simulink model "SensoSpoon_Control"  (R2026a)
settings: Solver=ode23t  StopTime=4  MaxStep=.001  RelTol=1e-4  AbsTol=1e-6
model workspace (MAT data in the model file):
  B(1).mass = 0.00253187337457
  B(1).com = [0.000428308261577; -3.33592024592e-19; -1.28078157724e-20]
  B(1).inertia = [7.38028719368e-08  -3.07478426256e-25  -1.32817521062e-25; -3.07478426256e-25  1.0653311692e-08  -5.88805898006e-25; -1.32817521062e-25  -5.88805898006e-25  7.14205635889e-08]
  B(2).mass = 0.046143480036
  B(2).com = [-0.0497444579629; 4.45344279178e-08; -0.0071916014832]
  B(2).inertia = [4.24326445066e-06  6.29131950445e-12  -4.63292057823e-06; 6.29131950445e-12  4.58365200995e-05  4.90790351694e-11; -4.63292057823e-06  4.90790351694e-11  4.73513997823e-05]
  B(3).mass = 0.011
  B(3).com = [0.049; -0.005; 0.006]
  B(3).inertia = [1.98e-07  0  0; 0  2.31e-07  0; 0  0  2.31e-07]
  B(4).mass = 0.0127643184343
  B(4).com = [0.0761622058383; 0.005; 0.006]
  B(4).inertia = [1.99984858239e-07  0  0; 0  2.24509835442e-06  0; 0  0  2.24509835442e-06]
  B(5).mass = 0.000712000026889
  B(5).com = [0; 0; 0]
  B(5).inertia = [3.56000013445e-10  0  0; 0  5.02701685652e-08  0; 0  0  5.02701685652e-08]
  B(6).mass = 0.000712000026889
  B(6).com = [0; 0; 0]
  B(6).inertia = [3.56000013445e-10  0  0; 0  5.02701685652e-08  0; 0  0  5.02701685652e-08]
  Bnom(1).mass = 0.00253187337457
  Bnom(1).com = [0.000428308261577; -3.33592024592e-19; -1.28078157724e-20]
  Bnom(1).inertia = [7.38028719368e-08  -3.07478426256e-25  -1.32817521062e-25; -3.07478426256e-25  1.0653311692e-08  -5.88805898006e-25; -1.32817521062e-25  -5.88805898006e-25  7.14205635889e-08]
  Bnom(2).mass = 0.043143480036
  Bnom(2).com = [-0.0486280291057; 4.76311480628e-08; -0.0069963183131]
  Bnom(2).inertia = [4.11170784507e-06  8.58555120438e-12  -4.48824336546e-06; 8.58555120438e-12  4.48215975922e-05  4.94803369061e-11; -4.48824336546e-06  4.94803369061e-11  4.62680338807e-05]
  Bnom(3).mass = 0.011
  Bnom(3).com = [0.049; -0.005; 0.006]
  Bnom(3).inertia = [1.98e-07  0  0; 0  2.31e-07  0; 0  0  2.31e-07]
  Bnom(4).mass = 0.0127643184343
  Bnom(4).com = [0.0761622058383; 0.005; 0.006]
  Bnom(4).inertia = [1.99984858239e-07  0  0; 0  2.24509835442e-06  0; 0  0  2.24509835442e-06]
  Bnom(5).mass = 0.000712000026889
  Bnom(5).com = [0; 0; 0]
  Bnom(5).inertia = [3.56000013445e-10  0  0; 0  5.02701685652e-08  0; 0  0  5.02701685652e-08]
  Bnom(6).mass = 0.000712000026889
  Bnom(6).com = [0; 0; 0]
  Bnom(6).inertia = [3.56000013445e-10  0  0; 0  5.02701685652e-08  0; 0  0  5.02701685652e-08]
  C.outer_hz = 800
  C.current_hz = 10000
  C.intent_filter = 'notch'
  C.notch_frequencies_Hz = [4 6 8 10 12]
  C.notch_bandwidth_Hz = 7
  C.intent_lead_s = 0.14
  C.intent_lead_pole_Hz = 1
  C.intent_rolloff_Hz = 10
  C.intent_hz = 1
  C.complement_hz = 0.05
  C.natural_hz = 35
  C.damping = 0.85
  C.integral_gain = 80
  C.current_kp = 0.8
  C.current_ki = 2000
  C.current_aw = 1500
  C.joint_limit = 0.244346095279
  C.reference_rate = 3.14159265359
  C.gyro_bias = [0.00347103685272; -0.00265540804355; 0.00180286392436; 0.00338772797741; -0.00268367652419; 0.00171822476761]
  C.accel_bias = [0.0499265864944; -0.0791463213806; 0.0291179813156; 0.0494836591873; -0.0770543876801; 0.0282725288544]
  C.current_quantum = 0.001708984375
  C.current_offset = [0.001; -0.001]
  C.current_noise_A = 0.0005
  C.power_window_s = 2
  C.seed = 1701
  C.name = 'simple_pid'
  C.intent_sos = [0.97325077265  -1.94554106429  0.97325077265  1  -1.94554106429  0.946501545301; 0.973256125668  -1.94435137935  0.973256125668  1  -1.94435137935  0.946512251336; 0.973263618882  -1.9426862109  0.973263618882  1  -1.9426862109  0.946527237765; 0.973273251283  -1.94054594933  0.973273251283  1  -1.94054594933  0.946546502566; 0.973285021571  -1.93793109639  0.973285021571  1  -1.93793109639  0.946570043141; 1.87620507603  -1.86838177621  0  1  -0.992176700178  0; 0.00146031630553  0.00292063261106  0.00146031630553  1  -1.88903307939  0.894874344617]
  H.revision = 'RCFlex_curved_neck_v17'
  H.total_length_mm = 271
  H.handle_mm = [168 30 24]
  H.bowl_mm = [62 40 12]
  H.bowl_tip_x_mm = -103
  H.bowl_widest_station_mm = 37.2
  H.bowl_front_width_mm = 28
  H.bowl_front_station_mm = 10.6338862458
  H.bowl_connection_width_mm = 10
  H.bowl_bottom_thickness_mm = 1.8
  H.bowl_measurement_x_mm = -65.8
  H.bowl_rim_z_mm = -4
  H.neck_length_mm = 31
  H.gimbal_mm = [25 33 19]
  H.pushrod_diameter_mm = 2
  H.physical_travel_deg = 15
  H.grip_x_mm = 65
  H.remote_center_x_mm = NaN
  H.equivalent_center_x_mm = 0
  H.shell_wall_mm = 1.4
  H.shell_x_mm = [0 18 35 55 80 100 130 150 160 168]
  H.shell_y_scale = [1.4 1.33333333333 1.2 1.1 1.08666666667 1.10666666667 1.14666666667 1.08666666667 0.8 0.133333333333]
  H.shell_z_scale = [1.75 1.66666666667 1.48333333333 1.16666666667 1.125 1.16666666667 1.25 1.16666666667 0.916666666667 0.166666666667]
  H.shell_center_z_mm = [0 0 1.5 4 6 6 6 6 6 6]
  H.ball_outer_radius_mm = 17
  H.ball_inner_radius_mm = 16.2
  H.ball_x_limits_mm = [-15.5 -3]
  H.bezel_outer_radius_mm = 21
  H.bezel_inner_radius_mm = 19.8
  H.bezel_x_limits_mm = [-16 0]
  H.front_cap_x_mm = 18
  H.front_rod_windows_mm = [-6.5  -2  9  18; 6.5  -2  9  18]
  H.bowl_wall_mm = 1.2
  H.vca_length_mm = 23.9
  H.vca_diameter_mm = 15.9
  H.vca_centers_mm = [55.5  -5  6; 87.5  5  6]
  H.vca_stroke_mm = 6.35
  H.vca_force_peak_N = 4.6
  H.vca_force_cont_N = 1.5
  H.vca_force_constant_N_A = 1.5
  H.steel_E_Pa = 200000000000
  H.flexure_pivot_parts = {'C-Flex B-10 x2 (pitch)', 'C-Flex D-10 x1 (roll)'}
  H.flexure_stiffness_Nm_rad = [0.00517884308057; 0.0116523969313]
  H.flexure_stiffness_tolerance = 0.1
  H.flexure_damping_Nms_rad = 0.0002
  H.flexure_cubic_ratio = 0
  H.fs = 1000
  H.duration = 20
  H.link.pivot = [0.012  0.012; -0.005  0.005; 0.0075  0.0075]
  H.link.mode = 'direct'
  H.link.attachment = [0.006  0.006; -0.0085  0.0085; -0.01  -0.01]
  H.link.slider_x = [0.03 0.03]
  H.link.slider_z = 0.006
  H.link.input_length = [0.0290559804515 0.0290559804515]
  H.link.output_length = 0
  H.coil_R_ohm = 4.6
  H.coil_L_H = 0.0008
  H.bus_voltage_V = 7.4
  H.current_limit_A = 1.5
  H.coil_alpha_K = 0.00393
  H.coil_mass_kg = 0.011
  H.motor_body_mass_kg = 0.017
  H.coil_continuous_power_W = 4.4
  H.shaft_side_load_N = 2.2
  H.driver_R_ohm = 0.7
  H.driver_pwm_hz = 20000
  H.driver_min_voltage_V = 4.5
  H.battery_capacity_Ah = 0.4
  H.battery_R_ohm = 0.15
  H.battery_mass_kg = 0.018
  H.battery_mm = [41 20 13]
  H.motor_part = 'Moticont GVCM-016-019-01M'
  H.driver_part = 'TI DRV8876PWPR'
  H.guide_friction_N = 0.03
  H.guide_viscous_Ns_m = 0.03
  H.imu_part = 'Bosch BMI270'
  H.imu_gyro_noise_dps_sqrtHz = 0.007
  H.imu_acc_noise_g_sqrtHz = 0.00016
  H.imu_gyro_offset_dps = 0.5
  H.imu_rate_hz = 800
  H.ambient_C = 25
  H.thermal_capacity_J_K = 8
  H.thermal_resistance_K_W = 18
  H.stop_stiffness_Nm_rad = 8
  H.stop_damping_Nms_rad = 0.025
  H.slider_stop_N_m = 10000
  H.slider_stop_Ns_m = 2
  H.food_mass_kg = 0.008
  H.sensor_seed = 1701
  Hnom.revision = 'RCFlex_curved_neck_v17'
  Hnom.total_length_mm = 271
  Hnom.handle_mm = [168 30 24]
  Hnom.bowl_mm = [62 40 12]
  Hnom.bowl_tip_x_mm = -103
  Hnom.bowl_widest_station_mm = 37.2
  Hnom.bowl_front_width_mm = 28
  Hnom.bowl_front_station_mm = 10.6338862458
  Hnom.bowl_connection_width_mm = 10
  Hnom.bowl_bottom_thickness_mm = 1.8
  Hnom.bowl_measurement_x_mm = -65.8
  Hnom.bowl_rim_z_mm = -4
  Hnom.neck_length_mm = 31
  Hnom.gimbal_mm = [25 33 19]
  Hnom.pushrod_diameter_mm = 2
  Hnom.physical_travel_deg = 15
  Hnom.grip_x_mm = 65
  Hnom.remote_center_x_mm = NaN
  Hnom.equivalent_center_x_mm = 0
  Hnom.shell_wall_mm = 1.4
  Hnom.shell_x_mm = [0 18 35 55 80 100 130 150 160 168]
  Hnom.shell_y_scale = [1.4 1.33333333333 1.2 1.1 1.08666666667 1.10666666667 1.14666666667 1.08666666667 0.8 0.133333333333]
  Hnom.shell_z_scale = [1.75 1.66666666667 1.48333333333 1.16666666667 1.125 1.16666666667 1.25 1.16666666667 0.916666666667 0.166666666667]
  Hnom.shell_center_z_mm = [0 0 1.5 4 6 6 6 6 6 6]
  Hnom.ball_outer_radius_mm = 17
  Hnom.ball_inner_radius_mm = 16.2
  Hnom.ball_x_limits_mm = [-15.5 -3]
  Hnom.bezel_outer_radius_mm = 21
  Hnom.bezel_inner_radius_mm = 19.8
  Hnom.bezel_x_limits_mm = [-16 0]
  Hnom.front_cap_x_mm = 18
  Hnom.front_rod_windows_mm = [-6.5  -2  9  18; 6.5  -2  9  18]
  Hnom.bowl_wall_mm = 1.2
  Hnom.vca_length_mm = 23.9
  Hnom.vca_diameter_mm = 15.9
  Hnom.vca_centers_mm = [55.5  -5  6; 87.5  5  6]
  Hnom.vca_stroke_mm = 6.35
  Hnom.vca_force_peak_N = 4.6
  Hnom.vca_force_cont_N = 1.5
  Hnom.vca_force_constant_N_A = 1.5
  Hnom.steel_E_Pa = 200000000000
  Hnom.flexure_pivot_parts = {'C-Flex B-10 x2 (pitch)', 'C-Flex D-10 x1 (roll)'}
  Hnom.flexure_stiffness_Nm_rad = [0.00517884308057; 0.0116523969313]
  Hnom.flexure_stiffness_tolerance = 0.1
  Hnom.flexure_damping_Nms_rad = 0.0002
  Hnom.flexure_cubic_ratio = 0
  Hnom.fs = 1000
  Hnom.duration = 20
  Hnom.link.pivot = [0.012  0.012; -0.005  0.005; 0.0075  0.0075]
  Hnom.link.mode = 'direct'
  Hnom.link.attachment = [0.006  0.006; -0.0085  0.0085; -0.01  -0.01]
  Hnom.link.slider_x = [0.03 0.03]
  Hnom.link.slider_z = 0.006
  Hnom.link.input_length = [0.0290559804515 0.0290559804515]
  Hnom.link.output_length = 0
  Hnom.coil_R_ohm = 4.6
  Hnom.coil_L_H = 0.0008
  Hnom.bus_voltage_V = 7.4
  Hnom.current_limit_A = 1.5
  Hnom.coil_alpha_K = 0.00393
  Hnom.coil_mass_kg = 0.011
  Hnom.motor_body_mass_kg = 0.017
  Hnom.coil_continuous_power_W = 4.4
  Hnom.shaft_side_load_N = 2.2
  Hnom.driver_R_ohm = 0.7
  Hnom.driver_pwm_hz = 20000
  Hnom.driver_min_voltage_V = 4.5
  Hnom.battery_capacity_Ah = 0.4
  Hnom.battery_R_ohm = 0.15
  Hnom.battery_mass_kg = 0.018
  Hnom.battery_mm = [41 20 13]
  Hnom.motor_part = 'Moticont GVCM-016-019-01M'
  Hnom.driver_part = 'TI DRV8876PWPR'
  Hnom.guide_friction_N = 0.03
  Hnom.guide_viscous_Ns_m = 0.03
  Hnom.imu_part = 'Bosch BMI270'
  Hnom.imu_gyro_noise_dps_sqrtHz = 0.007
  Hnom.imu_acc_noise_g_sqrtHz = 0.00016
  Hnom.imu_gyro_offset_dps = 0.5
  Hnom.imu_rate_hz = 800
  Hnom.ambient_C = 25
  Hnom.thermal_capacity_J_K = 8
  Hnom.thermal_resistance_K_W = 18
  Hnom.stop_stiffness_Nm_rad = 8
  Hnom.stop_damping_Nms_rad = 0.025
  Hnom.slider_stop_N_m = 10000
  Hnom.slider_stop_Ns_m = 2
  Hnom.food_mass_kg = 0.005
  base_motion = timeseries
  base_motion.Name = 'unnamed'
  base_motion.DataInfo = tsdata.datametadata
  base_motion.DataInfo.Interpolation = tsdata.interpolation
  base_motion.DataInfo.Interpolation.Fhandle : function handle (value not decoded)
  base_motion.DataInfo.Interpolation.Name = 'linear'
  base_motion.TimeInfo = tsdata.timemetadata
  base_motion.TimeInfo.Length = 80001
  base_motion.TimeInfo.DuplicateTimes = 0
  base_motion.TimeInfo.Time_ = [0 5e-05 0.0001 0.00015 0.0002 0.00025 0.0003 0.00035 0.0004 0.00045 0.0005 0.00055 ... (80001 elements, 80001x1)]
  base_motion.TimeInfo.Initialized = 1
  base_motion.QualityInfo = tsdata.qualmetadata
  base_motion.Data_ = [0 0 0 0 0 0 0 0 0 0 0 0 ... (1200015 elements, 80001x15)]
  mode = 'voltage'
  voltage_command = timeseries
  voltage_command.Name = 'unnamed'
  voltage_command.DataInfo = tsdata.datametadata
  voltage_command.DataInfo.Interpolation = tsdata.interpolation
  voltage_command.DataInfo.Interpolation.Fhandle : function handle (value not decoded)
  voltage_command.DataInfo.Interpolation.Name = 'linear'
  voltage_command.TimeInfo = tsdata.timemetadata
  voltage_command.TimeInfo.Length = 6001
  voltage_command.TimeInfo.DuplicateTimes = 0
  voltage_command.TimeInfo.Time_ = [0 0.001 0.002 0.003 0.004 0.005 0.006 0.007 0.008 0.009 0.01 0.011 ... (6001 elements, 6001x1)]
  voltage_command.TimeInfo.Initialized = 1
  voltage_command.QualityInfo = tsdata.qualmetadata
  voltage_command.Data_ = [0 0 0 0 0 0 0 0 0 0 0 0 ... (12002 elements, 6001x2)]
settings Model: Creator=tomli  LastModifiedBy=Aditya

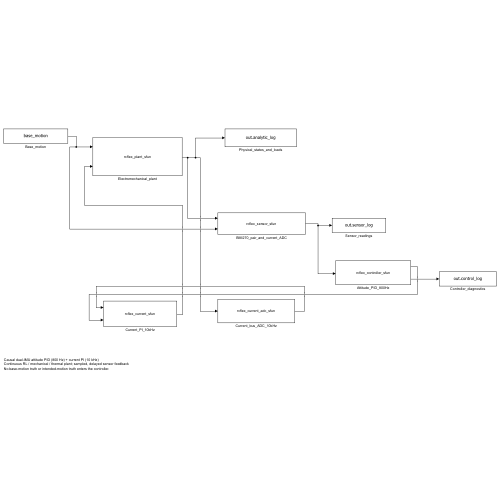
[thumbnail: Simulink's stored preview of the top-level diagram]
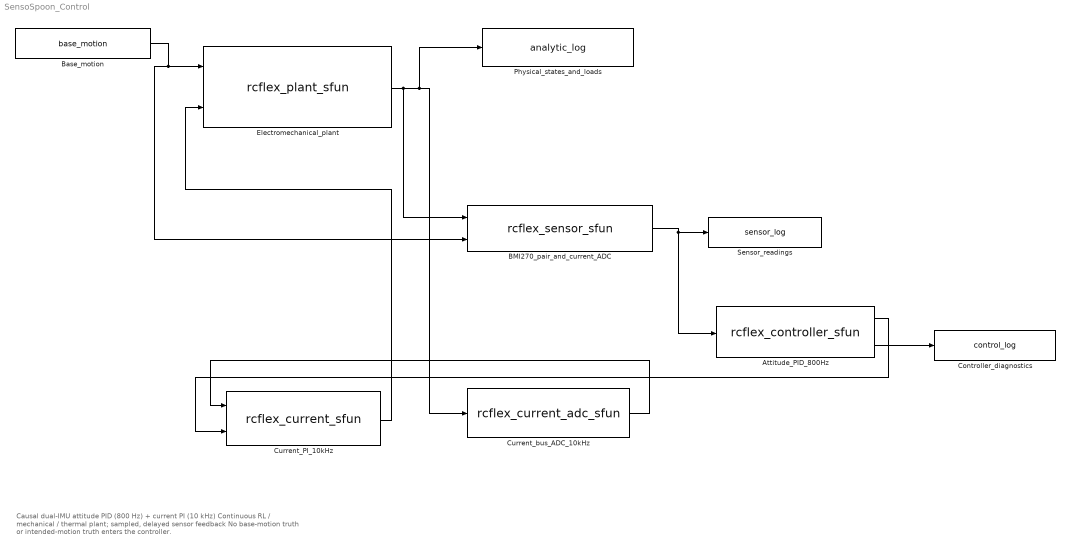
== system SensoSpoon_Control ==
  note: Causal dual-IMU attitude PID (800 Hz) + current PI (10 kHz)
      | Continuous RL / mechanical / thermal plant; sampled, delayed sensor feedback
      | No base-motion truth or intended-motion truth enters the controller.
  Attitude_PID_800Hz : M-S-Function  FunctionName=rcflex_controller_sfun  Parameters=Hnom,Bnom,C
  BMI270_pair_and_current_ADC : M-S-Function  FunctionName=rcflex_sensor_sfun  Parameters=H
  Base_motion : FromWorkspace  VariableName=base_motion
  Controller_diagnostics : ToWorkspace  VariableName=control_log  SaveFormat=Timeseries  SampleTime=-1
  Current_PI_10kHz : M-S-Function  FunctionName=rcflex_current_sfun  Parameters=Hnom,C
  Current_bus_ADC_10kHz : M-S-Function  FunctionName=rcflex_current_adc_sfun  Parameters=H,C
  Electromechanical_plant : M-S-Function  FunctionName=rcflex_plant_sfun  Parameters=H,B,mode
  Physical_states_and_loads : ToWorkspace  VariableName=analytic_log  SaveFormat=Timeseries  SampleTime=-1
  Sensor_readings : ToWorkspace  VariableName=sensor_log  SaveFormat=Timeseries  SampleTime=-1
  wires:
  Base_motion/1 -> BMI270_pair_and_current_ADC/2, Electromechanical_plant/1
  Electromechanical_plant/1 -> Physical_states_and_loads/1, Current_bus_ADC_10kHz/1, BMI270_pair_and_current_ADC/1
  BMI270_pair_and_current_ADC/1 -> Sensor_readings/1, Attitude_PID_800Hz/1
  Attitude_PID_800Hz/1 -> Current_PI_10kHz/2
  Attitude_PID_800Hz/2 -> Controller_diagnostics/1
  Current_bus_ADC_10kHz/1 -> Current_PI_10kHz/1
  Current_PI_10kHz/1 -> Electromechanical_plant/2
